simulink model "mvc"  (R2016b)
settings: Solver=VariableStepAuto  StartTime=0.0  StopTime=.5  RelTol=1e-3
libraries: powerlib x37, powerlib_meascontrol x19, simulink x8
settings Model: Creator=Dell  LastModifiedBy=Dell

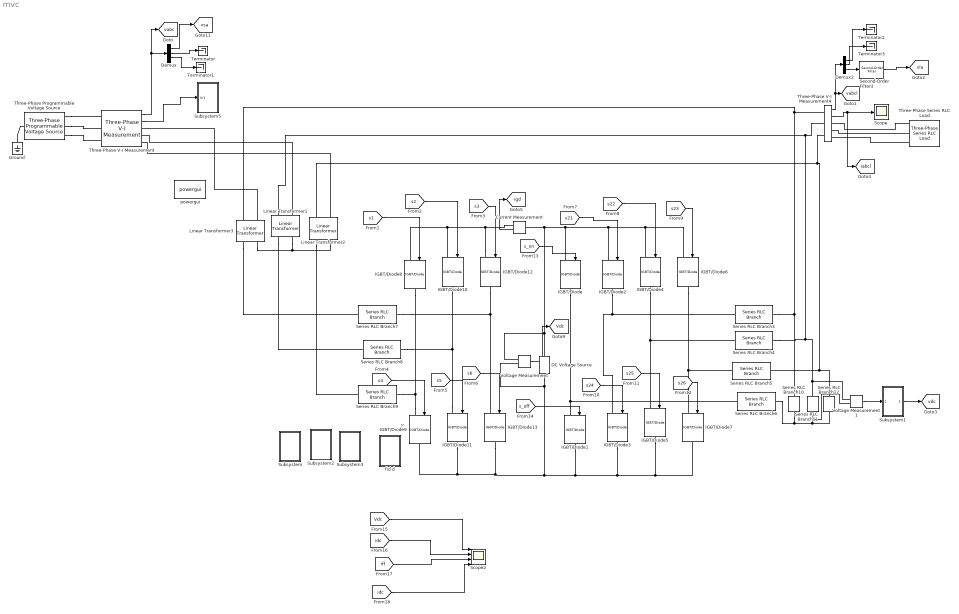
== system mvc ==
  note: rc
  Current Measurement : powerlib/Measurements/Current Measurement  PhasorSimulation=off  OutputType=Complex  PSBequivalent=0
  DC Voltage Source : powerlib/Electrical Sources/DC Voltage Source  Amplitude=400  Measurements=None
  Demux : Demux  Outputs=3
  Demux2 : Demux  Outputs=3
  Ground : powerlib/Elements/Ground  LConnTagsString=a
  IGBT/Diode{,1..13} (14 alike) : powerlib/Power Electronics/IGBT//Diode  Ron=1e-3  Rs=1e5  Cs=inf  Measurements=off
  Linear Transformer1 : powerlib/Elements/Linear Transformer  UNITS=pu  NominalPower=[ 3e3 50 ]  winding1="[ 3e3 0.002  0.08 ]"  winding2="[ 3e3  0.002  0.08 ]"  ThreeWindings=off  winding3=[ 315e3 0.002 0.08 ]  RmLm=[ 500 500 ]  Measurements=None  DataType=off
  Linear Transformer2 : powerlib/Elements/Linear Transformer  UNITS=pu  NominalPower=[ 3e3 50 ]  winding1="[ 3e3 0.002  0.08 ]"  winding2="[ 3e3  0.002  0.08 ]"  ThreeWindings=off  winding3=[ 315e3 0.002 0.08 ]  RmLm=[ 500 500 ]  Measurements=None  DataType=off
  Linear Transformer3 : powerlib/Elements/Linear Transformer  UNITS=pu  NominalPower=[ 3e3 50 ]  winding1="[ 3e3 0.002  0.08 ]"  winding2="[ 3e3  0.002  0.08 ]"  ThreeWindings=off  winding3=[ 315e3 0.002 0.08 ]  RmLm=[ 500 500 ]  Measurements=None  DataType=off
  Scope : Scope
  Scope2 : Scope  NumInputPorts=4
  Second-Order Filter3 : powerlib_meascontrol/Filters/Second-Order Filter  FilterType=Lowpass  Fo=50  Zeta=0.707  Ts=0  Initialize=on  Vac_Init="[0,  0,  50]"  Vdc_Init=0  PlotResponse=off  FreqRange=[0, 500, 1]
  Series RLC Branch10 : powerlib/Elements/Series RLC Branch  LConnTagsString=__new0  RConnTagsString=__new0  BranchType=C  Resistance=1  Inductance=1e-3  SetiL0=off  InitialCurrent=0  Capacitance=1e-6  Setx0=off  InitialVoltage=0  Measurements=None
  Series RLC Branch11 : powerlib/Elements/Series RLC Branch  LConnTagsString=__new0  RConnTagsString=__new0  BranchType=C  Resistance=1  Inductance=1e-3  SetiL0=off  InitialCurrent=0  Capacitance=1e-6  Setx0=off  InitialVoltage=0  Measurements=None
  Series RLC Branch12 : powerlib/Elements/Series RLC Branch  LConnTagsString=__new0  RConnTagsString=__new0  BranchType=C  Resistance=1  Inductance=1e-3  SetiL0=off  InitialCurrent=0  Capacitance=1e-6  Setx0=off  InitialVoltage=0  Measurements=None
  Series RLC Branch{3..9} (7 alike) : powerlib/Elements/Series RLC Branch  LConnTagsString=__new0  RConnTagsString=__new0  BranchType=RL  Resistance=1  Inductance=1e-3  SetiL0=off  InitialCurrent=0  Capacitance=1e-6  Setx0=off  InitialVoltage=0  Measurements=None
  Subsystem : Subsystem
  Subsystem1 : Subsystem
  Subsystem2 : Subsystem
  Subsystem3 : Subsystem
  Subsystem5 : Subsystem
  Terminator{,1..3} (4 alike) : Terminator
  Three-Phase Programmable Voltage Source : powerlib/Electrical Sources/Three-Phase Programmable Voltage Source  PositiveSequence="[100  0 50]"  VariationEntity=Amplitude  VariationType=Table of time-amplitude pairs  VariationTypeAlt=Step  VariationStep=0.5  VariationRate=10  VariationMagnitude=0.3  VariationFrequency=2  VariationTiming=[1 2]  VariationPhaseA=off  Amplitudes=[1 0.82 0.82 1.0]  TimeValues=[0 0.2 0.3 0.4]  HarmonicGeneration=off  HarmonicA=[3 0.2 -25 0]  HarmonicB=[2 0.15 35 2]  Timing="[0.05  3]"  BusType=swing  Pref=0  Qref=0  Qmin=-inf  Qmax=inf
  Three-Phase Series RLC Load : powerlib/Elements/Three-Phase Series RLC Load  LConnTagsString=A|B|C  Configuration=Y (grounded)  NominalVoltage=1000  Vabc=[1e3 1e3 1e3]  Vabcp=[1e3 1e3 1e3]  NominalFrequency=50  UnbalancedPower=off  ActivePower=10e3  InductivePower=100  CapacitivePower=100  Pabc=[10e3 9e3 11e3]  QLabc=[100 90 110]  QCabc=[100 90 110]  Pabcp=[10e3 9e3 11e3]  QLabcp=[100 90 110]  QCabcp=[100 90 110]  Measurements=None  LoadType=constant Z
  Three-Phase V-I Measurement : powerlib/Measurements/Three-Phase V-I Measurement  VoltageMeasurement=phase-to-phase  SetLabelV=off  LabelV=Vabc  Vpu=off  VpuLL=off  CurrentMeasurement=yes  SetLabelI=off  LabelI=Iabc  Ipu=off  Pbase=100e6  Vbase=500e3  OutputType=Complex  PhasorSimulation=off  PSBequivalent=0
  Three-Phase V-I Measurement4 : powerlib/Measurements/Three-Phase V-I Measurement  VoltageMeasurement=phase-to-phase  SetLabelV=off  LabelV=Vabcl  Vpu=off  VpuLL=off  CurrentMeasurement=yes  SetLabelI=off  LabelI=Iabcl  Ipu=off  Pbase=100e6  Vbase=500e3  OutputType=Complex  PhasorSimulation=off  PSBequivalent=0
  Voltage Measurement : powerlib/Measurements/Voltage Measurement  PhasorSimulation=off  OutputType=Complex  PSBequivalent=0
  Voltage Measurement1 : powerlib/Measurements/Voltage Measurement  PhasorSimulation=off  OutputType=Complex  PSBequivalent=0
  fid d : Subsystem
  powergui : powerlib/powergui  Priority=1  SimulationMode=Discrete  SolverType=Tustin/Backward Euler (TBE)  SampleTime=50e-6  frequency=60  SPID=off  DisableSnubberDevices=off  DisableRonSwitches=off  DisableVfSwitches=off  SwTol=0  DisplayEquations=off  Interpol=off  ExternalGateDelay=off  methode=off  Ts=10  FunctionMessages=off  echomessages=off  HookPort=off  EnableUseOfTLC=off  x0status=blocks  frequencyindice=0  Pbase=100e6  ErrMax=1e-4  Iterations=50  UnitsV=kV  UnitsW=MW  buscounter=0  RestoreLinks=warning  ResistiveCurrentMeasurement=off  Frange=[0:2:500]  Ylog=off  Xlog=on  ShowGrid=off  save=off  variable=ZData  structure=0  ZoomFFT=off  StartTime=0.0  cycles=1  DisplayStyle=1  fundamental=60  FreqAxis=off  MaxFrequency=1000  frequencyindicesteady=1  RmsSteady=1  display=off
  tag scope: Vdc=global, iabcl=global, igd=global, vabc=global, vabcl=global, vdc=global, vla=global, vsa=global
  wires:
  Three-Phase V-I Measurement/2 -> Subsystem5/1(In1)
  [s1] -> IGBT/Diode8/1
  [s2] -> IGBT/Diode10/1
  [s3] -> IGBT/Diode12/1
  [s4] -> IGBT/Diode9/1
  [s5] -> IGBT/Diode11/1
  [s6] -> IGBT/Diode13/1
  [s21] -> IGBT/Diode2/1
  [s22] -> IGBT/Diode4/1
  [s23] -> IGBT/Diode6/1
  [s24] -> IGBT/Diode3/1
  [s25] -> IGBT/Diode5/1
  [s26] -> IGBT/Diode7/1
  [s_on] -> IGBT/Diode/1
  [s_off] -> IGBT/Diode1/1
  Voltage Measurement/1 -> [Vdc]
  Three-Phase V-I Measurement/1 -> [vabc], Demux/1
  Demux/1 -> [vsa]
  [Vdc] -> Scope2/1
  [idc] -> Scope2/2
  [iff] -> Scope2/3
  [idc] -> Scope2/4
  Three-Phase V-I Measurement4/2 -> [iabcl], Scope/1
  Three-Phase V-I Measurement4/1 -> [vabcl], Demux2/1
  Demux2/3 -> Second-Order Filter3/1
  Second-Order Filter3/1 -> [vla]
  Voltage Measurement1/1 -> Subsystem1/1(In1)
  Subsystem1/1(Out1) -> [vdc]
  Demux/2 -> Terminator/1
  Demux/3 -> Terminator1/1
  Demux2/1 -> Terminator2/1
  Demux2/2 -> Terminator3/1
  Current Measurement/1 -> [igd]
  connections:
  Linear Transformer3/RConn2 -- Linear Transformer1/RConn2 -- Linear Transformer2/RConn2
  Series RLC Branch6/LConn1 -- IGBT/Diode1/LConn1 -- IGBT/Diode/RConn1
  Series RLC Branch3/LConn1 -- IGBT/Diode2/RConn1 -- IGBT/Diode3/LConn1
  Series RLC Branch4/LConn1 -- IGBT/Diode4/RConn1 -- IGBT/Diode5/LConn1
  Series RLC Branch5/LConn1 -- IGBT/Diode6/RConn1 -- IGBT/Diode7/LConn1
  IGBT/Diode3/RConn1 -- IGBT/Diode13/RConn1 -- IGBT/Diode11/RConn1 -- IGBT/Diode9/RConn1 -- DC Voltage Source/LConn1 -- Voltage Measurement/LConn2 -- IGBT/Diode1/RConn1 -- IGBT/Diode7/RConn1 -- IGBT/Diode5/RConn1
  IGBT/Diode12/LConn1 -- Current Measurement/RConn1 -- IGBT/Diode8/LConn1 -- IGBT/Diode10/LConn1
  Series RLC Branch7/RConn1 -- IGBT/Diode12/RConn1 -- IGBT/Diode13/LConn1
  IGBT/Diode11/LConn1 -- IGBT/Diode10/RConn1 -- Series RLC Branch8/RConn1
  IGBT/Diode9/LConn1 -- IGBT/Diode8/RConn1 -- Series RLC Branch9/RConn1
  Series RLC Branch11/LConn1 -- Voltage Measurement1/LConn1 -- Series RLC Branch4/RConn1 -- Linear Transformer1/LConn1 -- Three-Phase V-I Measurement4/LConn2
  Three-Phase V-I Measurement4/LConn3 -- Series RLC Branch12/LConn1 -- Series RLC Branch5/RConn1 -- Linear Transformer2/LConn1
  Series RLC Branch12/RConn1 -- Voltage Measurement1/LConn2 -- Series RLC Branch11/RConn1 -- Series RLC Branch10/RConn1 -- Series RLC Branch6/RConn1
  Series RLC Branch10/LConn1 -- Linear Transformer3/LConn1 -- Three-Phase V-I Measurement4/LConn1 -- Series RLC Branch3/RConn1
  Linear Transformer2/LConn2 -- Three-Phase V-I Measurement/RConn3
  Linear Transformer3/LConn2 -- Three-Phase V-I Measurement/RConn1
  Three-Phase Series RLC Load/LConn1 -- Three-Phase V-I Measurement4/RConn1
  Three-Phase Programmable Voltage Source/RConn2 -- Three-Phase V-I Measurement/LConn2
  Three-Phase Series RLC Load/LConn2 -- Three-Phase V-I Measurement4/RConn2
  Three-Phase Series RLC Load/LConn3 -- Three-Phase V-I Measurement4/RConn3
  Linear Transformer3/RConn1 -- Series RLC Branch7/LConn1
  Linear Transformer1/RConn1 -- Series RLC Branch8/LConn1
  Linear Transformer2/RConn1 -- Series RLC Branch9/LConn1
  Linear Transformer1/LConn2 -- Three-Phase V-I Measurement/RConn2
  Three-Phase Programmable Voltage Source/RConn1 -- Three-Phase V-I Measurement/LConn1
  Three-Phase Programmable Voltage Source/RConn3 -- Three-Phase V-I Measurement/LConn3
  Ground/LConn1 -- Three-Phase Programmable Voltage Source/LConn1
  IGBT/Diode2/LConn1 -- IGBT/Diode/LConn1 -- Current Measurement/LConn1 -- DC Voltage Source/RConn1 -- Voltage Measurement/LConn1 -- IGBT/Diode6/LConn1 -- IGBT/Diode4/LConn1

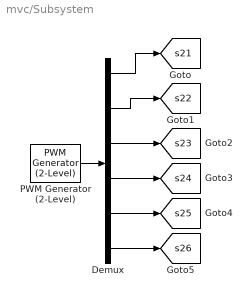
== system mvc/Subsystem ==
  Demux : Demux  Outputs=6
  PWM Generator (2-Level) : powerlib_meascontrol/Pulse & Signal Generators/PWM Generator (2-Level)  ModulatorType=Three-phase bridge (6 pulses)  ModulatorMode=Unsynchronized  Fc=27*60  Pc=90  nF=27  MinMax="[ -1  1 ]"  SamplingTechnique=Natural  ModulatingSignals=on  m=0.8  Freq=50  Phase=0  Ts=0  ShowCarrierOutport=off
  tag scope: s21=global, s22=global, s23=global, s24=global, s25=global, s26=global
  wires:
  PWM Generator (2-Level)/1 -> Demux/1
  Demux/1 -> [s21]
  Demux/2 -> [s22]
  Demux/3 -> [s23]
  Demux/4 -> [s24]
  Demux/5 -> [s25]
  Demux/6 -> [s26]

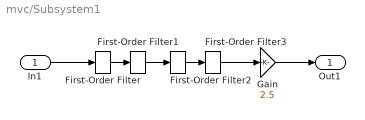
== system mvc/Subsystem1 ==
  In1 : Inport
  First-Order Filter{,1..3} (4 alike) : powerlib_meascontrol/Filters/First-Order Filter  FilterType=Lowpass  Tc=10e-3  Ts=0  Initialize=on  Vac_Init=[0, 0, 60]  Vdc_Init=0  PlotResponse=off  FreqRange="[0,  200,  1]"
  Gain : Gain  Gain=2.5
  Out1 : Outport
  wires:
  In1/1 -> First-Order Filter/1
  First-Order Filter/1 -> First-Order Filter1/1
  First-Order Filter1/1 -> First-Order Filter2/1
  First-Order Filter3/1 -> Gain/1
  First-Order Filter2/1 -> First-Order Filter3/1
  Gain/1 -> Out1/1

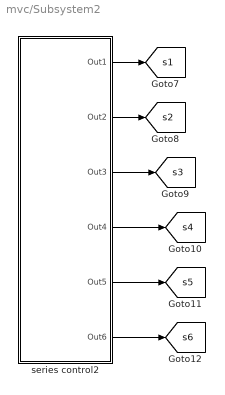
== system mvc/Subsystem2 ==
  series control2 : Subsystem
  tag scope: s1=global, s2=global, s3=global, s4=global, s5=global, s6=global
  wires:
  series control2/1(Out1) -> [s1]
  series control2/2(Out2) -> [s2]
  series control2/3(Out3) -> [s3]
  series control2/4(Out4) -> [s4]
  series control2/5(Out5) -> [s5]
  series control2/6(Out6) -> [s6]

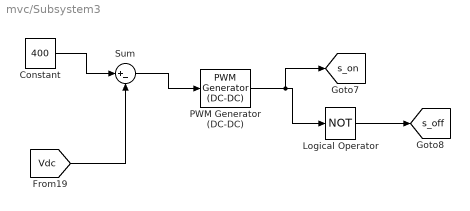
== system mvc/Subsystem3 ==
  Constant : Constant  Value=400
  Logical Operator : Logic  Operator=NOT  AllPortsSameDT=off  OutDataTypeStr=boolean
  PWM Generator (DC-DC) : powerlib_meascontrol/Pulse & Signal Generators/PWM Generator (DC-DC)  Fsw=5000  Ts=0
  Sum : Sum  Inputs=|+-
  tag scope: s_off=global, s_on=global
  wires:
  Sum/1 -> PWM Generator (DC-DC)/1
  PWM Generator (DC-DC)/1 -> [s_on], Logical Operator/1
  [Vdc] -> Sum/2
  Logical Operator/1 -> [s_off]
  Constant/1 -> Sum/1

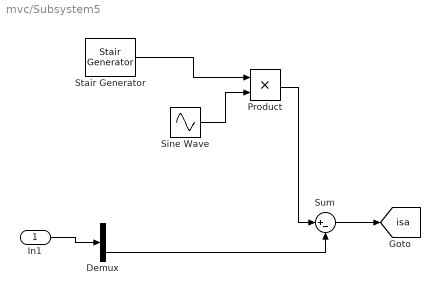
== system mvc/Subsystem5 ==
  In1 : Inport
  Demux : Demux  Outputs=3
  Product : Product
  Sine Wave : Sin  Amplitude=20  Frequency=2*pi*50  SampleTime=0
  Stair Generator : powerlib_meascontrol/Pulse & Signal Generators/Stair Generator  t=[0 0.2 0.3 0.4]  e=[1 1.6 1.6 1.0]  Ts=0
  Sum : Sum  Inputs=|+-
  tag scope: isa=global
  wires:
  Sum/1 -> [isa]
  Demux/3 -> Sum/2
  In1/1 -> Demux/1
  Product/1 -> Sum/1
  Stair Generator/1 -> Product/1
  Sine Wave/1 -> Product/2

== system mvc/fid d ==
  Scope : Scope  NumInputPorts=2
  Scope2 : Scope  NumInputPorts=4
  wires:
  [vsa] -> Scope/2, Scope2/2
  [vla] -> Scope2/3
  [Vdc] -> Scope2/1
  [isa] -> Scope/1, Scope2/4

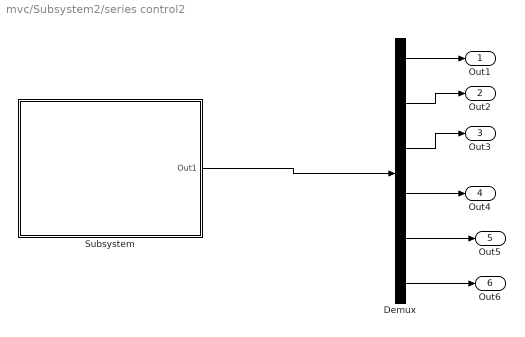
== system mvc/Subsystem2/series control2 ==
  Demux : Demux  Outputs=6
  Subsystem : Subsystem
  Out1 : Outport
  Out2 : Outport  Port=2
  Out3 : Outport  Port=3
  Out4 : Outport  Port=4
  Out5 : Outport  Port=5
  Out6 : Outport  Port=6
  wires:
  Demux/1 -> Out1/1
  Demux/2 -> Out2/1
  Demux/3 -> Out3/1
  Demux/4 -> Out4/1
  Demux/5 -> Out5/1
  Demux/6 -> Out6/1
  Subsystem/1(Out1) -> Demux/1

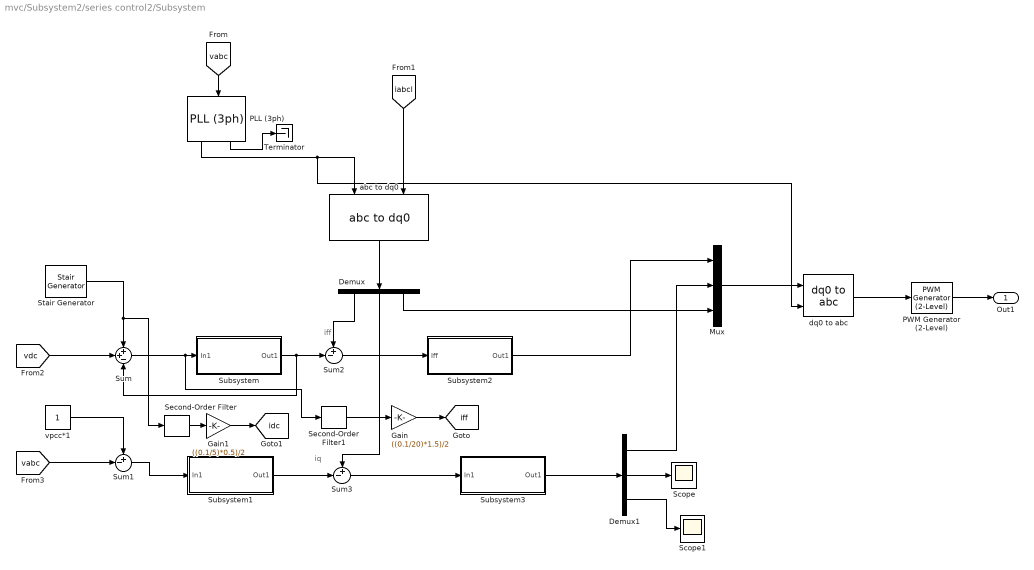
== system mvc/Subsystem2/series control2/Subsystem ==
  note: iq
  note: iff
  Demux : Demux  Outputs=3
  Demux1 : Demux  Outputs=3
  Gain : Gain  Gain=((0.1/20)*1.5)/2
  Gain1 : Gain  Gain=((0.1/5)*0.5)/2
  Mux : Mux  Inputs=3
  PLL (3ph) : powerlib_meascontrol/PLL/PLL (3ph)  Fmin=45  Par_Init=[0, 60]  ParK=[180, 3200, 1]  TcD=1e-4  MaxRateChangeFreq=12  FilterCutOffFreq=25  Ts=0  AGC=on
  PWM Generator (2-Level) : powerlib_meascontrol/Pulse & Signal Generators/PWM Generator (2-Level)  ModulatorType=Three-phase bridge (6 pulses)  ModulatorMode=Unsynchronized  Fc=27*60  Pc=90  nF=27  MinMax="[ -1  1 ]"  SamplingTechnique=Natural  ModulatingSignals=off  m=0.8  Freq=60  Phase=0  Ts=0  ShowCarrierOutport=off
  Scope : Scope
  Scope1 : Scope
  Second-Order Filter : powerlib_meascontrol/Filters/Second-Order Filter  FilterType=Lowpass  Fo=50  Zeta=0.707  Ts=0  Initialize=on  Vac_Init="[0,  0,  60]"  Vdc_Init=0  PlotResponse=off  FreqRange=[0, 500, 1]
  Second-Order Filter1 : powerlib_meascontrol/Filters/Second-Order Filter  FilterType=Lowpass  Fo=50  Zeta=0.707  Ts=0  Initialize=on  Vac_Init="[0,  0,  60]"  Vdc_Init=0  PlotResponse=off  FreqRange=[0, 500, 1]
  Stair Generator : powerlib_meascontrol/Pulse & Signal Generators/Stair Generator  t=[0 0.2 0.3 0.4]  e=[400,390, 400, 400]  Ts=0
  Subsystem : Subsystem
  Subsystem1 : Subsystem
  Subsystem2 : Subsystem
  Subsystem3 : Subsystem
  Sum : Sum  Inputs=++-
  Sum1 : Sum  Inputs=+-|
  Sum2 : Sum  Inputs=+-|
  Sum3 : Sum  Inputs=+-|
  Terminator : Terminator
  abc to dq0 : powerlib_meascontrol/Transformations/abc to dq0  Alignment=90 degrees behind phase A axis
  dq0 to abc : powerlib_meascontrol/Transformations/dq0 to abc  Alignment=90 degrees behind phase A axis
  vpcc*1 : Constant
  Out1 : Outport
  tag scope: idc=global, iff=global
  wires:
  [vdc] -> Sum/2
  Stair Generator/1 -> Second-Order Filter/1, Sum/1
  [vabc] -> Sum1/2
  vpcc*1/1 -> Sum1/1
  [vabc] -> PLL (3ph)/1
  [iabcl] -> abc to dq0/1
  PLL (3ph)/2 -> dq0 to abc/2, abc to dq0/2
  abc to dq0/1 -> Demux/1
  Sum/1 -> Second-Order Filter1/1, Subsystem/1(In1)
  Sum1/1 -> Subsystem1/1(In1)
  Subsystem/1(Out1) -> Sum/3, Sum2/2
  Demux/1 -> Sum2/1
  Subsystem1/1(Out1) -> Sum3/2
  Demux/2 -> Sum3/1
  Demux/3 -> Mux/3
  Sum3/1 -> Subsystem3/1(In1)
  Sum2/1 -> Subsystem2/1(Iff)
  Mux/1 -> dq0 to abc/1
  dq0 to abc/1 -> PWM Generator (2-Level)/1
  PWM Generator (2-Level)/1 -> Out1/1
  Subsystem3/1(Out1) -> Demux1/1
  Demux1/1 -> Mux/2
  Demux1/2 -> Scope/1
  Demux1/3 -> Scope1/1
  Subsystem2/1(Out1) -> Mux/1
  Second-Order Filter/1 -> Gain1/1
  Second-Order Filter1/1 -> Gain/1
  Gain/1 -> [iff]
  Gain1/1 -> [idc]
  PLL (3ph)/1 -> Terminator/1

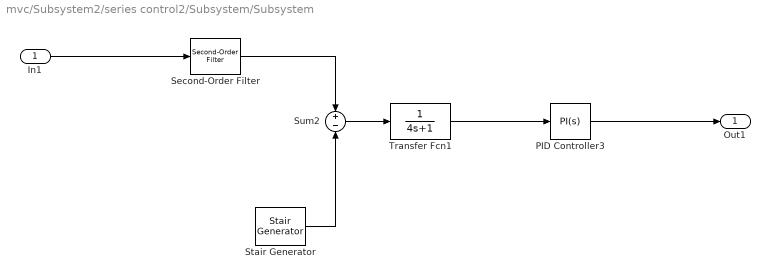
== system mvc/Subsystem2/series control2/Subsystem/Subsystem ==
  In1 : Inport
  PID Controller3 : simulink/Continuous/PID Controller  Controller=PI  TimeDomain=Continuous-time  SampleTime=-1  IntegratorMethod=Forward Euler  FilterMethod=Forward Euler  Form=Parallel  UseFilter=on  ControllerParametersSource=internal  P=1  I=1  D=0  N=100  InitialConditionSource=internal  InitialConditionForIntegrator=0  InitialConditionForFilter=0  ExternalReset=none  LimitOutput=off  UpperSaturationLimit=inf  LowerSaturationLimit=-inf  LinearizeAsGain=on  AntiWindupMode=none  Kb=1  TrackingMode=off  Kt=1  PParamMin=[]  PParamMax=[]  IParamMin=[]  IParamMax=[]  DParamMin=[]  DParamMax=[]  NParamMin=[]  NParamMax=[]  KbParamMin=[]  KbParamMax=[]  KtParamMin=[]  KtParamMax=[]  POutMin=[]  POutMax=[]  IOutMin=[]  IOutMax=[]  DOutMin=[]  DOutMax=[]  NOutMin=[]  NOutMax=[]  KbOutMin=[]  KbOutMax=[]  KtOutMin=[]  KtOutMax=[]  IntegratorOutMin=[]  IntegratorOutMax=[]  FilterOutMin=[]  FilterOutMax=[]  SumOutMin=[]  SumOutMax=[]  SumI1OutMin=[]  SumI1OutMax=[]  SumI2OutMin=[]  SumI2OutMax=[]  SumI3OutMin=[]  SumI3OutMax=[]  SumDOutMin=[]  SumDOutMax=[]  SaturationOutMin=[]  SaturationOutMax=[]  IntegratorContinuousStateAttributes=''  IntegratorStateMustResolveToSignalObject=off  IntegratorRTWStateStorageClass=Auto  FilterContinuousStateAttributes=''  FilterStateMustResolveToSignalObject=off  FilterRTWStateStorageClass=Auto  DifferentiatorICPrevScaledInput=0  DifferentiatorOutMin=[]  DifferentiatorOutMax=[]
  Second-Order Filter : powerlib_meascontrol/Filters/Second-Order Filter  FilterType=Lowpass  Fo=50  Zeta=0.707  Ts=0  Initialize=on  Vac_Init="[0,  0,  60]"  Vdc_Init=0  PlotResponse=off  FreqRange=[0, 500, 1]
  Stair Generator : powerlib_meascontrol/Pulse & Signal Generators/Stair Generator  t=[0 0.2 0.3 0.4]  e=[1,2.1, 1, 1]  Ts=0
  Sum2 : Sum  Inputs=+-
  Transfer Fcn1 : TransferFcn  Denominator=[4 1]
  Out1 : Outport
  wires:
  In1/1 -> Second-Order Filter/1
  Sum2/1 -> Transfer Fcn1/1
  Transfer Fcn1/1 -> PID Controller3/1
  Second-Order Filter/1 -> Sum2/1
  PID Controller3/1 -> Out1/1
  Stair Generator/1 -> Sum2/2

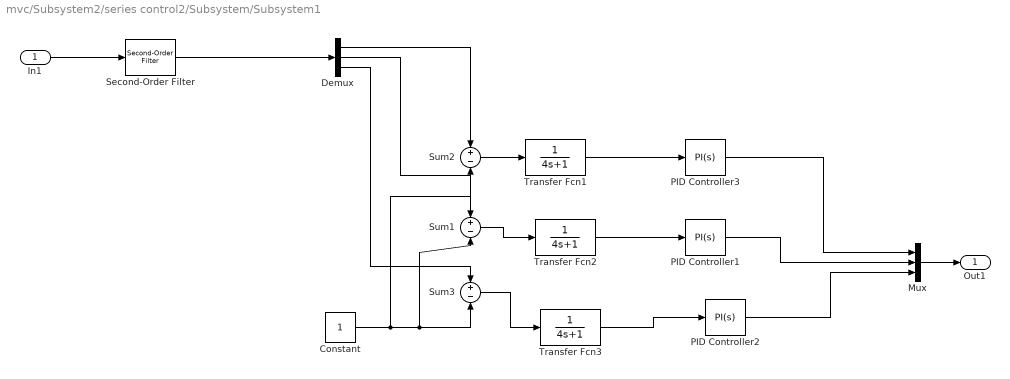
== system mvc/Subsystem2/series control2/Subsystem/Subsystem1 ==
  In1 : Inport
  Constant : Constant
  Demux : Demux  Outputs=3
  Mux : Mux  Inputs=3
  PID Controller1 : simulink/Continuous/PID Controller  Controller=PI  TimeDomain=Continuous-time  SampleTime=-1  IntegratorMethod=Forward Euler  FilterMethod=Forward Euler  Form=Parallel  UseFilter=on  ControllerParametersSource=internal  P=1  I=1  D=0  N=100  InitialConditionSource=internal  InitialConditionForIntegrator=0  InitialConditionForFilter=0  ExternalReset=none  LimitOutput=off  UpperSaturationLimit=inf  LowerSaturationLimit=-inf  LinearizeAsGain=on  AntiWindupMode=none  Kb=1  TrackingMode=off  Kt=1  PParamMin=[]  PParamMax=[]  IParamMin=[]  IParamMax=[]  DParamMin=[]  DParamMax=[]  NParamMin=[]  NParamMax=[]  KbParamMin=[]  KbParamMax=[]  KtParamMin=[]  KtParamMax=[]  POutMin=[]  POutMax=[]  IOutMin=[]  IOutMax=[]  DOutMin=[]  DOutMax=[]  NOutMin=[]  NOutMax=[]  KbOutMin=[]  KbOutMax=[]  KtOutMin=[]  KtOutMax=[]  IntegratorOutMin=[]  IntegratorOutMax=[]  FilterOutMin=[]  FilterOutMax=[]  SumOutMin=[]  SumOutMax=[]  SumI1OutMin=[]  SumI1OutMax=[]  SumI2OutMin=[]  SumI2OutMax=[]  SumI3OutMin=[]  SumI3OutMax=[]  SumDOutMin=[]  SumDOutMax=[]  SaturationOutMin=[]  SaturationOutMax=[]  IntegratorContinuousStateAttributes=''  IntegratorStateMustResolveToSignalObject=off  IntegratorRTWStateStorageClass=Auto  FilterContinuousStateAttributes=''  FilterStateMustResolveToSignalObject=off  FilterRTWStateStorageClass=Auto  DifferentiatorICPrevScaledInput=0  DifferentiatorOutMin=[]  DifferentiatorOutMax=[]
  PID Controller2 : simulink/Continuous/PID Controller  Controller=PI  TimeDomain=Continuous-time  SampleTime=-1  IntegratorMethod=Forward Euler  FilterMethod=Forward Euler  Form=Parallel  UseFilter=on  ControllerParametersSource=internal  P=1  I=1  D=0  N=100  InitialConditionSource=internal  InitialConditionForIntegrator=0  InitialConditionForFilter=0  ExternalReset=none  LimitOutput=off  UpperSaturationLimit=inf  LowerSaturationLimit=-inf  LinearizeAsGain=on  AntiWindupMode=none  Kb=1  TrackingMode=off  Kt=1  PParamMin=[]  PParamMax=[]  IParamMin=[]  IParamMax=[]  DParamMin=[]  DParamMax=[]  NParamMin=[]  NParamMax=[]  KbParamMin=[]  KbParamMax=[]  KtParamMin=[]  KtParamMax=[]  POutMin=[]  POutMax=[]  IOutMin=[]  IOutMax=[]  DOutMin=[]  DOutMax=[]  NOutMin=[]  NOutMax=[]  KbOutMin=[]  KbOutMax=[]  KtOutMin=[]  KtOutMax=[]  IntegratorOutMin=[]  IntegratorOutMax=[]  FilterOutMin=[]  FilterOutMax=[]  SumOutMin=[]  SumOutMax=[]  SumI1OutMin=[]  SumI1OutMax=[]  SumI2OutMin=[]  SumI2OutMax=[]  SumI3OutMin=[]  SumI3OutMax=[]  SumDOutMin=[]  SumDOutMax=[]  SaturationOutMin=[]  SaturationOutMax=[]  IntegratorContinuousStateAttributes=''  IntegratorStateMustResolveToSignalObject=off  IntegratorRTWStateStorageClass=Auto  FilterContinuousStateAttributes=''  FilterStateMustResolveToSignalObject=off  FilterRTWStateStorageClass=Auto  DifferentiatorICPrevScaledInput=0  DifferentiatorOutMin=[]  DifferentiatorOutMax=[]
  PID Controller3 : simulink/Continuous/PID Controller  Controller=PI  TimeDomain=Continuous-time  SampleTime=-1  IntegratorMethod=Forward Euler  FilterMethod=Forward Euler  Form=Parallel  UseFilter=on  ControllerParametersSource=internal  P=1  I=1  D=0  N=100  InitialConditionSource=internal  InitialConditionForIntegrator=0  InitialConditionForFilter=0  ExternalReset=none  LimitOutput=off  UpperSaturationLimit=inf  LowerSaturationLimit=-inf  LinearizeAsGain=on  AntiWindupMode=none  Kb=1  TrackingMode=off  Kt=1  PParamMin=[]  PParamMax=[]  IParamMin=[]  IParamMax=[]  DParamMin=[]  DParamMax=[]  NParamMin=[]  NParamMax=[]  KbParamMin=[]  KbParamMax=[]  KtParamMin=[]  KtParamMax=[]  POutMin=[]  POutMax=[]  IOutMin=[]  IOutMax=[]  DOutMin=[]  DOutMax=[]  NOutMin=[]  NOutMax=[]  KbOutMin=[]  KbOutMax=[]  KtOutMin=[]  KtOutMax=[]  IntegratorOutMin=[]  IntegratorOutMax=[]  FilterOutMin=[]  FilterOutMax=[]  SumOutMin=[]  SumOutMax=[]  SumI1OutMin=[]  SumI1OutMax=[]  SumI2OutMin=[]  SumI2OutMax=[]  SumI3OutMin=[]  SumI3OutMax=[]  SumDOutMin=[]  SumDOutMax=[]  SaturationOutMin=[]  SaturationOutMax=[]  IntegratorContinuousStateAttributes=''  IntegratorStateMustResolveToSignalObject=off  IntegratorRTWStateStorageClass=Auto  FilterContinuousStateAttributes=''  FilterStateMustResolveToSignalObject=off  FilterRTWStateStorageClass=Auto  DifferentiatorICPrevScaledInput=0  DifferentiatorOutMin=[]  DifferentiatorOutMax=[]
  Second-Order Filter : powerlib_meascontrol/Filters/Second-Order Filter  FilterType=Lowpass  Fo=50  Zeta=0.707  Ts=0  Initialize=on  Vac_Init="[0,  0,  60]"  Vdc_Init=0  PlotResponse=off  FreqRange=[0, 500, 1]
  Sum1 : Sum  Inputs=+-
  Sum2 : Sum  Inputs=+-
  Sum3 : Sum  Inputs=+-
  Transfer Fcn1 : TransferFcn  Denominator=[4 1]
  Transfer Fcn2 : TransferFcn  Denominator=[4 1]
  Transfer Fcn3 : TransferFcn  Denominator=[4 1]
  Out1 : Outport
  wires:
  PID Controller3/1 -> Mux/1
  Second-Order Filter/1 -> Demux/1
  Transfer Fcn1/1 -> PID Controller3/1
  Sum2/1 -> Transfer Fcn1/1
  In1/1 -> Second-Order Filter/1
  Transfer Fcn2/1 -> PID Controller1/1
  Transfer Fcn3/1 -> PID Controller2/1
  PID Controller1/1 -> Mux/2
  PID Controller2/1 -> Mux/3
  Mux/1 -> Out1/1
  Demux/1 -> Sum2/1
  Sum1/1 -> Transfer Fcn2/1
  Sum3/1 -> Transfer Fcn3/1
  Demux/2 -> Sum1/1
  Demux/3 -> Sum3/1
  Constant/1 -> Sum2/2, Sum1/2, Sum3/2

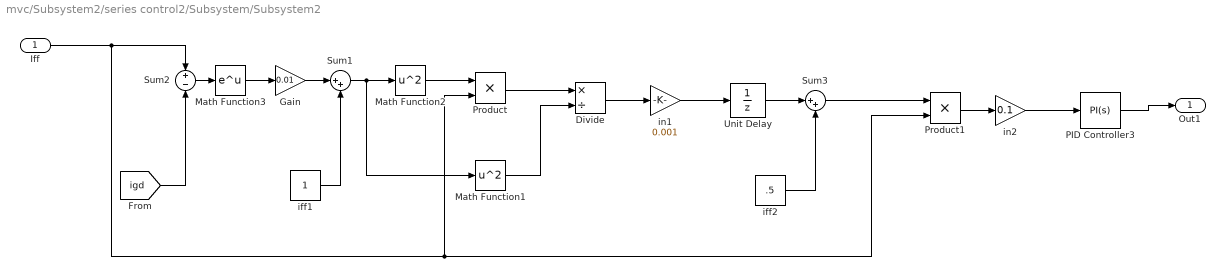
== system mvc/Subsystem2/series control2/Subsystem/Subsystem2 ==
  Iff : Inport
  Divide : Product  Inputs=*/
  Gain : Gain  Gain=0.01
  Math Function1 : Math  Operator=square  SaturateOnIntegerOverflow=on
  Math Function2 : Math  Operator=square  SaturateOnIntegerOverflow=on
  Math Function3 : Math  SaturateOnIntegerOverflow=on
  PID Controller3 : simulink/Continuous/PID Controller  Controller=PI  TimeDomain=Continuous-time  SampleTime=-1  IntegratorMethod=Forward Euler  FilterMethod=Forward Euler  Form=Parallel  UseFilter=on  ControllerParametersSource=internal  P=1  I=1  D=0  N=100  InitialConditionSource=internal  InitialConditionForIntegrator=0  InitialConditionForFilter=0  ExternalReset=none  LimitOutput=off  UpperSaturationLimit=inf  LowerSaturationLimit=-inf  LinearizeAsGain=on  AntiWindupMode=none  Kb=1  TrackingMode=off  Kt=1  PParamMin=[]  PParamMax=[]  IParamMin=[]  IParamMax=[]  DParamMin=[]  DParamMax=[]  NParamMin=[]  NParamMax=[]  KbParamMin=[]  KbParamMax=[]  KtParamMin=[]  KtParamMax=[]  POutMin=[]  POutMax=[]  IOutMin=[]  IOutMax=[]  DOutMin=[]  DOutMax=[]  NOutMin=[]  NOutMax=[]  KbOutMin=[]  KbOutMax=[]  KtOutMin=[]  KtOutMax=[]  IntegratorOutMin=[]  IntegratorOutMax=[]  FilterOutMin=[]  FilterOutMax=[]  SumOutMin=[]  SumOutMax=[]  SumI1OutMin=[]  SumI1OutMax=[]  SumI2OutMin=[]  SumI2OutMax=[]  SumI3OutMin=[]  SumI3OutMax=[]  SumDOutMin=[]  SumDOutMax=[]  SaturationOutMin=[]  SaturationOutMax=[]  IntegratorContinuousStateAttributes=''  IntegratorStateMustResolveToSignalObject=off  IntegratorRTWStateStorageClass=Auto  FilterContinuousStateAttributes=''  FilterStateMustResolveToSignalObject=off  FilterRTWStateStorageClass=Auto  DifferentiatorICPrevScaledInput=0  DifferentiatorOutMin=[]  DifferentiatorOutMax=[]
  Product : Product
  Product1 : Product
  Sum1 : Sum  Inputs=|++
  Sum2 : Sum  Inputs=+-
  Sum3 : Sum  Inputs=|++
  Unit Delay : UnitDelay  SampleTime=-1
  iff1 : Constant
  iff2 : Constant  Value=.5
  in1 : Gain  Gain=0.001
  in2 : Gain  Gain=0.1
  Out1 : Outport
  wires:
  [igd] -> Sum2/2
  PID Controller3/1 -> Out1/1
  Sum2/1 -> Math Function3/1
  Math Function3/1 -> Gain/1
  Gain/1 -> Sum1/1
  iff1/1 -> Sum1/2
  Sum1/1 -> Math Function1/1, Math Function2/1
  Math Function2/1 -> Product/1
  Iff/1 -> Sum2/1, Product/2, Product1/2
  Product/1 -> Divide/1
  Math Function1/1 -> Divide/2
  Divide/1 -> in1/1
  in1/1 -> Unit Delay/1
  Unit Delay/1 -> Sum3/1
  iff2/1 -> Sum3/2
  Sum3/1 -> Product1/1
  Product1/1 -> in2/1
  in2/1 -> PID Controller3/1

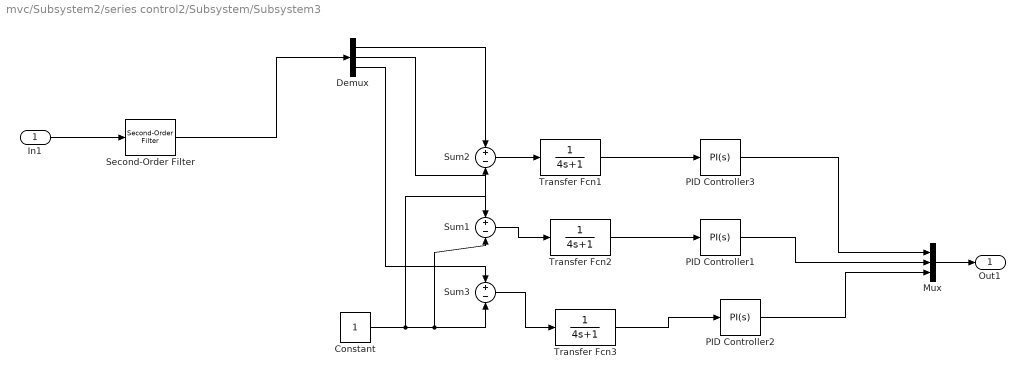
== system mvc/Subsystem2/series control2/Subsystem/Subsystem3 ==
  In1 : Inport
  Constant : Constant
  Demux : Demux  Outputs=3
  Mux : Mux  Inputs=3
  PID Controller1 : simulink/Continuous/PID Controller  Controller=PI  TimeDomain=Continuous-time  SampleTime=-1  IntegratorMethod=Forward Euler  FilterMethod=Forward Euler  Form=Parallel  UseFilter=on  ControllerParametersSource=internal  P=1  I=1  D=0  N=100  InitialConditionSource=internal  InitialConditionForIntegrator=0  InitialConditionForFilter=0  ExternalReset=none  LimitOutput=off  UpperSaturationLimit=inf  LowerSaturationLimit=-inf  LinearizeAsGain=on  AntiWindupMode=none  Kb=1  TrackingMode=off  Kt=1  PParamMin=[]  PParamMax=[]  IParamMin=[]  IParamMax=[]  DParamMin=[]  DParamMax=[]  NParamMin=[]  NParamMax=[]  KbParamMin=[]  KbParamMax=[]  KtParamMin=[]  KtParamMax=[]  POutMin=[]  POutMax=[]  IOutMin=[]  IOutMax=[]  DOutMin=[]  DOutMax=[]  NOutMin=[]  NOutMax=[]  KbOutMin=[]  KbOutMax=[]  KtOutMin=[]  KtOutMax=[]  IntegratorOutMin=[]  IntegratorOutMax=[]  FilterOutMin=[]  FilterOutMax=[]  SumOutMin=[]  SumOutMax=[]  SumI1OutMin=[]  SumI1OutMax=[]  SumI2OutMin=[]  SumI2OutMax=[]  SumI3OutMin=[]  SumI3OutMax=[]  SumDOutMin=[]  SumDOutMax=[]  SaturationOutMin=[]  SaturationOutMax=[]  IntegratorContinuousStateAttributes=''  IntegratorStateMustResolveToSignalObject=off  IntegratorRTWStateStorageClass=Auto  FilterContinuousStateAttributes=''  FilterStateMustResolveToSignalObject=off  FilterRTWStateStorageClass=Auto  DifferentiatorICPrevScaledInput=0  DifferentiatorOutMin=[]  DifferentiatorOutMax=[]
  PID Controller2 : simulink/Continuous/PID Controller  Controller=PI  TimeDomain=Continuous-time  SampleTime=-1  IntegratorMethod=Forward Euler  FilterMethod=Forward Euler  Form=Parallel  UseFilter=on  ControllerParametersSource=internal  P=1  I=1  D=0  N=100  InitialConditionSource=internal  InitialConditionForIntegrator=0  InitialConditionForFilter=0  ExternalReset=none  LimitOutput=off  UpperSaturationLimit=inf  LowerSaturationLimit=-inf  LinearizeAsGain=on  AntiWindupMode=none  Kb=1  TrackingMode=off  Kt=1  PParamMin=[]  PParamMax=[]  IParamMin=[]  IParamMax=[]  DParamMin=[]  DParamMax=[]  NParamMin=[]  NParamMax=[]  KbParamMin=[]  KbParamMax=[]  KtParamMin=[]  KtParamMax=[]  POutMin=[]  POutMax=[]  IOutMin=[]  IOutMax=[]  DOutMin=[]  DOutMax=[]  NOutMin=[]  NOutMax=[]  KbOutMin=[]  KbOutMax=[]  KtOutMin=[]  KtOutMax=[]  IntegratorOutMin=[]  IntegratorOutMax=[]  FilterOutMin=[]  FilterOutMax=[]  SumOutMin=[]  SumOutMax=[]  SumI1OutMin=[]  SumI1OutMax=[]  SumI2OutMin=[]  SumI2OutMax=[]  SumI3OutMin=[]  SumI3OutMax=[]  SumDOutMin=[]  SumDOutMax=[]  SaturationOutMin=[]  SaturationOutMax=[]  IntegratorContinuousStateAttributes=''  IntegratorStateMustResolveToSignalObject=off  IntegratorRTWStateStorageClass=Auto  FilterContinuousStateAttributes=''  FilterStateMustResolveToSignalObject=off  FilterRTWStateStorageClass=Auto  DifferentiatorICPrevScaledInput=0  DifferentiatorOutMin=[]  DifferentiatorOutMax=[]
  PID Controller3 : simulink/Continuous/PID Controller  Controller=PI  TimeDomain=Continuous-time  SampleTime=-1  IntegratorMethod=Forward Euler  FilterMethod=Forward Euler  Form=Parallel  UseFilter=on  ControllerParametersSource=internal  P=1  I=1  D=0  N=100  InitialConditionSource=internal  InitialConditionForIntegrator=0  InitialConditionForFilter=0  ExternalReset=none  LimitOutput=off  UpperSaturationLimit=inf  LowerSaturationLimit=-inf  LinearizeAsGain=on  AntiWindupMode=none  Kb=1  TrackingMode=off  Kt=1  PParamMin=[]  PParamMax=[]  IParamMin=[]  IParamMax=[]  DParamMin=[]  DParamMax=[]  NParamMin=[]  NParamMax=[]  KbParamMin=[]  KbParamMax=[]  KtParamMin=[]  KtParamMax=[]  POutMin=[]  POutMax=[]  IOutMin=[]  IOutMax=[]  DOutMin=[]  DOutMax=[]  NOutMin=[]  NOutMax=[]  KbOutMin=[]  KbOutMax=[]  KtOutMin=[]  KtOutMax=[]  IntegratorOutMin=[]  IntegratorOutMax=[]  FilterOutMin=[]  FilterOutMax=[]  SumOutMin=[]  SumOutMax=[]  SumI1OutMin=[]  SumI1OutMax=[]  SumI2OutMin=[]  SumI2OutMax=[]  SumI3OutMin=[]  SumI3OutMax=[]  SumDOutMin=[]  SumDOutMax=[]  SaturationOutMin=[]  SaturationOutMax=[]  IntegratorContinuousStateAttributes=''  IntegratorStateMustResolveToSignalObject=off  IntegratorRTWStateStorageClass=Auto  FilterContinuousStateAttributes=''  FilterStateMustResolveToSignalObject=off  FilterRTWStateStorageClass=Auto  DifferentiatorICPrevScaledInput=0  DifferentiatorOutMin=[]  DifferentiatorOutMax=[]
  Second-Order Filter : powerlib_meascontrol/Filters/Second-Order Filter  FilterType=Lowpass  Fo=50  Zeta=0.707  Ts=0  Initialize=on  Vac_Init="[0,  0,  60]"  Vdc_Init=0  PlotResponse=off  FreqRange=[0, 500, 1]
  Sum1 : Sum  Inputs=+-
  Sum2 : Sum  Inputs=+-
  Sum3 : Sum  Inputs=+-
  Transfer Fcn1 : TransferFcn  Denominator=[4 1]
  Transfer Fcn2 : TransferFcn  Denominator=[4 1]
  Transfer Fcn3 : TransferFcn  Denominator=[4 1]
  Out1 : Outport
  wires:
  PID Controller3/1 -> Mux/1
  Second-Order Filter/1 -> Demux/1
  Transfer Fcn1/1 -> PID Controller3/1
  Sum2/1 -> Transfer Fcn1/1
  In1/1 -> Second-Order Filter/1
  Transfer Fcn2/1 -> PID Controller1/1
  Transfer Fcn3/1 -> PID Controller2/1
  PID Controller1/1 -> Mux/2
  PID Controller2/1 -> Mux/3
  Mux/1 -> Out1/1
  Demux/1 -> Sum2/1
  Sum1/1 -> Transfer Fcn2/1
  Sum3/1 -> Transfer Fcn3/1
  Demux/2 -> Sum1/1
  Demux/3 -> Sum3/1
  Constant/1 -> Sum2/2, Sum1/2, Sum3/2
